simulink model "SupplyMonitor"  (R2024a)
settings: Solver=FixedStepDiscrete  StartTime=0.0  StopTime=10  FixedStep=0.01  RelTol=1e-3
model workspace (MAT data in the model file):
  CurrentInvalid_cycles = Simulink.Parameter
  CurrentInvalid_cycles.Value = 20
  CurrentInvalid_cycles.Complexity = 'real'
  CurrentInvalid_cycles.Dimensions = [1 1]
  CurrentInvalid_cycles.DataType = 'uint8'
  MinCurrentTime_cycles = Simulink.Parameter
  MinCurrentTime_cycles.Value = 20
  MinCurrentTime_cycles.Complexity = 'real'
  MinCurrentTime_cycles.Dimensions = [1 1]
  MinCurrentTime_cycles.DataType = 'uint8'
  MinCurrent_mA = Simulink.Parameter
  MinCurrent_mA.Value = 100
  MinCurrent_mA.Complexity = 'real'
  MinCurrent_mA.Dimensions = [1 1]
  MinCurrent_mA.DataType = 'single'
  OverloadHyst_mA = Simulink.Parameter
  OverloadHyst_mA.Value = 200
  OverloadHyst_mA.Complexity = 'real'
  OverloadHyst_mA.Dimensions = [1 1]
  OverloadHyst_mA.DataType = 'single'
  OverloadThd_mA = Simulink.Parameter
  OverloadThd_mA.Value = 1280
  OverloadThd_mA.Complexity = 'real'
  OverloadThd_mA.Dimensions = [1 1]
  OverloadThd_mA.DataType = 'single'
  SupplyCurrentFilter = Simulink.Parameter
  SupplyCurrentFilter.Value = 0.0078125
  SupplyCurrentFilter.Complexity = 'real'
  SupplyCurrentFilter.Dimensions = [1 1]
  SupplyCurrentFilter.DataType = 'single'
  SupplyCurrentGain = Simulink.Parameter
  SupplyCurrentGain.Value = 1
  SupplyCurrentGain.Complexity = 'real'
  SupplyCurrentGain.Dimensions = [1 1]
  SupplyCurrentGain.DataType = 'single'
values from neighbouring files (symbols this model uses):
  CurrentInvalid_cycles = 20    [SupplyMonitor_data.m]
  MinCurrent_mA = 100    [SupplyMonitor_data.m]
  MinCurrentTime_cycles = 20    [SupplyMonitor_data.m]
  OverloadHyst_mA = 200    [SupplyMonitor_data.m]
  OverloadThd_mA = 1280    [SupplyMonitor_data.m]
  SupplyCurrentFilter = 0.0078125    [SupplyMonitor_data.m]
  SupplyCurrentGain = 1.0    (= 1)    [SupplyMonitor_data.m]
undefined symbols (not defined in the file or in its folder): QLF_OK
Description:
  | 48-V-Versorgung: Strom filtern, Ueberlast mit Hysterese, LIMIT-Leitung
settings Model: ParameterArgumentNames=SupplyCurrentFilter,SupplyCurrentGain,OverloadThd_mA,OverloadHyst_mA,MinCurrent_mA,MinCurrentTime_cycles,CurrentInvalid_cycles  Creator=danie  LastModifiedBy=danie
settings OptimizationCC: DefaultParameterBehavior=Inlined  EnhancedBackFolding=on  PassReuseOutputArgsAs=Individual arguments  ZeroExternalMemoryAtStartup=off  ZeroInternalMemoryAtStartup=off  OptimizeBlockOrder=speed  DifferentSizesBufferReuse=on  OptimizationCustomize=off  EfficientTunableParamExpr=on
settings DebuggingCC: ParameterTunabilityLossMsg=error
settings HardwareCC: ProdBitPerPointer=32  ProdBitPerSizeT=32  ProdBitPerPtrDiffT=32  ProdLargestAtomicInteger=Long  ProdLargestAtomicFloat=Double  ProdWordSize=32  ProdLongLongMode=on  ProdHWDeviceType=ARM Compatible->ARM Cortex-M
settings SFSimCC: MATLABDynamicMemAlloc=off
settings RTWCC: Description=AUTOSAR  SystemTargetFile=autosar.tlc  GenCodeOnly=on  GenerateMakefile=off  TemplateMakefile=ert_default_tmf  DataTypeReplacement=CDataTypesFixedWidth
settings CodeAppCC: ForceParamTrailComments=on  IgnoreCustomStorageClasses=off  MaxIdLength=63  OperatorAnnotations=on  SimulinkDataObjDesc=on  SFDataObjDesc=on  InsertBlockDesc=on
settings STFCustomTargetCC: MultiwordLength=256  ParMdlRefBuildCompliant=on  CompOptLevelCompliant=on  IncludeMdlTerminateFcn=off  CombineOutputUpdateFcns=on  SuppressErrorStatus=on  ERTCustomFileBanners=on  SupportNonFinite=off  SupportComplex=off  SupportContinuousTime=off  SupportNonInlinedSFcns=off  RemoveResetFunc=on  MATLABClassNameForMDSCustomization=Simulink.SoftwareTarget.ERTCustomization  AutosarCompliant=on  GRTInterface=off  LookupTableObjectStructAxisOrder=2,1,3,4,...  LUTObjectStructOrderEvenSpacing=Size,Table,Breakpoints  SystemTargetFile=autosar.tlc
settings ERTTargetCC: TargetLangStandard=C99 (ISO)  ConcurrentExecutionCompliant=off  IncludeMdlTerminateFcn=off  SuppressErrorStatus=on  SupportNonFinite=off  SupportComplex=off  ModelStepFunctionPrototypeControlCompliant=off  CPPClassGenCompliant=off  AutosarCompliant=on  LookupTableObjectStructAxisOrder=2,1,3,4,...  LUTObjectStructOrderEvenSpacing=Size,Table,Breakpoints  InlinedParameterPlacement=NonHierarchical  ERTCustomFileTemplate=example_file_process.tlc  BooleanTrueId=TRUE  BooleanFalseId=FALSE

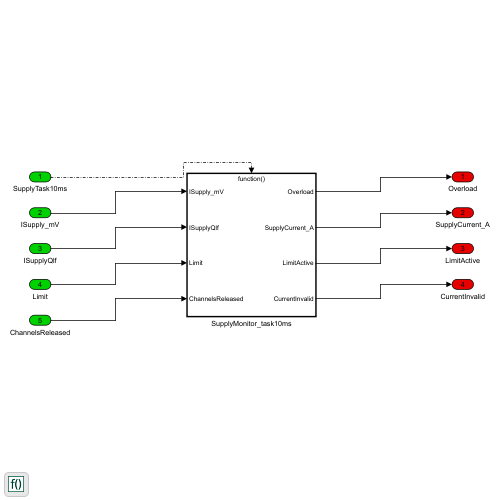
[thumbnail: Simulink's stored preview of the top-level diagram]
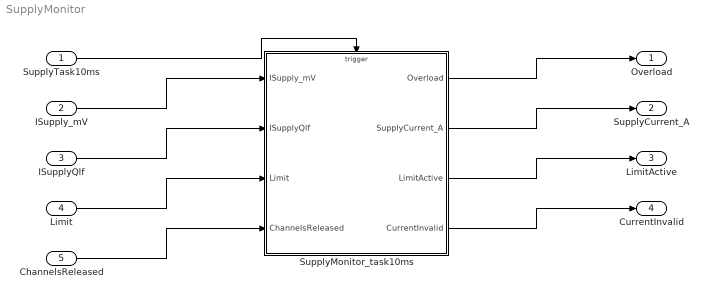
== system SupplyMonitor ==
  SupplyTask10ms : Inport  SampleTime=0.01  OutputFunctionCall=on
  ISupply_mV : Inport  Port=2  OutDataTypeStr=uint32  PortDimensions=1
  ISupplyQlf : Inport  Port=3  OutDataTypeStr=uint8  PortDimensions=1
  Limit : Inport  Port=4  OutDataTypeStr=boolean  PortDimensions=1
  ChannelsReleased : Inport  Port=5  OutDataTypeStr=boolean  PortDimensions=1
  SupplyMonitor_task10ms : Subsystem  TreatAsAtomicUnit=on
  Overload : Outport  OutDataTypeStr=boolean  PortDimensions=1
  SupplyCurrent_A : Outport  Port=2  OutDataTypeStr=single  PortDimensions=1
  LimitActive : Outport  Port=3  OutDataTypeStr=boolean  PortDimensions=1
  CurrentInvalid : Outport  Port=4  OutDataTypeStr=boolean  PortDimensions=1
  wires:
  SupplyTask10ms/1 -> SupplyMonitor_task10ms/Trigger
  ISupply_mV/1 -> SupplyMonitor_task10ms/1(ISupply_mV)
  ISupplyQlf/1 -> SupplyMonitor_task10ms/2(ISupplyQlf)
  Limit/1 -> SupplyMonitor_task10ms/3(Limit)
  ChannelsReleased/1 -> SupplyMonitor_task10ms/4(ChannelsReleased)
  SupplyMonitor_task10ms/1(Overload) -> Overload/1
  SupplyMonitor_task10ms/2(SupplyCurrent_A) -> SupplyCurrent_A/1
  SupplyMonitor_task10ms/3(LimitActive) -> LimitActive/1
  SupplyMonitor_task10ms/4(CurrentInvalid) -> CurrentInvalid/1

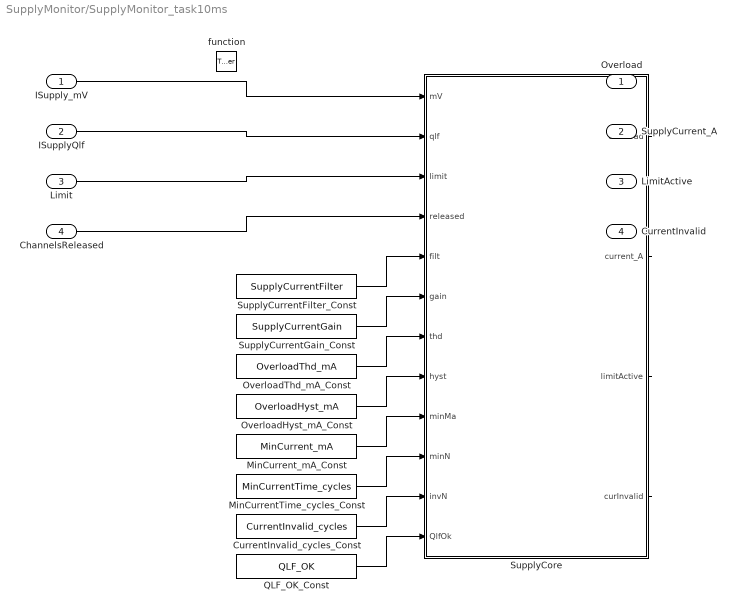
== system SupplyMonitor/SupplyMonitor_task10ms ==
  ISupply_mV : Inport
  ISupplyQlf : Inport  Port=2
  Limit : Inport  Port=3
  ChannelsReleased : Inport  Port=4
  function : TriggerPort  TriggerType=function-call  VariantControl=(inherit)  SampleTimeType=periodic  SampleTime=0.01
  CurrentInvalid_cycles_Const : Constant  Value=CurrentInvalid_cycles  OutDataTypeStr=uint8
  MinCurrentTime_cycles_Const : Constant  Value=MinCurrentTime_cycles  OutDataTypeStr=uint8
  MinCurrent_mA_Const : Constant  Value=MinCurrent_mA  OutDataTypeStr=single
  OverloadHyst_mA_Const : Constant  Value=OverloadHyst_mA  OutDataTypeStr=single
  OverloadThd_mA_Const : Constant  Value=OverloadThd_mA  OutDataTypeStr=single
  QLF_OK_Const : Constant  Value=QLF_OK  OutDataTypeStr=uint8
  SupplyCore : MATLAB Function  TreatAsAtomicUnit=on
  SupplyCurrentFilter_Const : Constant  Value=SupplyCurrentFilter  OutDataTypeStr=single
  SupplyCurrentGain_Const : Constant  Value=SupplyCurrentGain  OutDataTypeStr=single
  Overload : Outport
  SupplyCurrent_A : Outport  Port=2
  LimitActive : Outport  Port=3
  CurrentInvalid : Outport  Port=4
  wires:
  ISupply_mV/1 -> SupplyCore/1(mV)
  ISupplyQlf/1 -> SupplyCore/2(qlf)
  Limit/1 -> SupplyCore/3(limit)
  ChannelsReleased/1 -> SupplyCore/4(released)
  SupplyCurrentFilter_Const/1 -> SupplyCore/5(filt)
  SupplyCurrentGain_Const/1 -> SupplyCore/6(gain)
  OverloadThd_mA_Const/1 -> SupplyCore/7(thd)
  OverloadHyst_mA_Const/1 -> SupplyCore/8(hyst)
  MinCurrent_mA_Const/1 -> SupplyCore/9(minMa)
  MinCurrentTime_cycles_Const/1 -> SupplyCore/10(minN)
  CurrentInvalid_cycles_Const/1 -> SupplyCore/11(invN)
  QLF_OK_Const/1 -> SupplyCore/12(QlfOk)
  SupplyCore/1(overload) -> Overload/1
  SupplyCore/2(current_A) -> SupplyCurrent_A/1
  SupplyCore/3(limitActive) -> LimitActive/1
  SupplyCore/4(curInvalid) -> CurrentInvalid/1

== matlab function SupplyMonitor/SupplyMonitor_task10ms/SupplyCore ==
  data: mV input; overload output; qlf input; limit input; released input; filt input; gain input; thd input; hyst input; minMa input; minN input; invN input; QlfOk input; current_A output; limitActive output; curInvalid output
function [overload, current_A, limitActive, curInvalid] = SupplyCore(mV, qlf, limit, released, filt, gain, thd, hyst, minMa, minN, invN, QlfOk)
%SUPPLYCORE 48 V supply current filter, overload with hysteresis (see SupplyMonitor_create.m).
%#codegen
persistent y ovl bad low
if isempty(y)
    y = single(0);      % filtered current [mA]
    ovl = false;
    bad = uint8(0);     % invalid samples in a row (saturating)
    low = uint8(0);     % implausibly low valid samples in a row with a channel released (saturating)
end
if qlf == QlfOk
    sample = single(mV) * gain;
    y = y + filt * (sample - y);
    bad = uint8(0);
    if released && (sample < minMa)
        if low < uint8(255)
            low = low + uint8(1);
        end
    else
        low = uint8(0);
    end
elseif bad < uint8(255)
    bad = bad + uint8(1);
end
if ~released
    low = uint8(0);
end
if y > thd
    ovl = true;
elseif y < thd - hyst
    ovl = false;
end
overload = ovl;
c = y * single(0.001);
if c > single(65.535)
    c = single(65.535);
end
current_A = c;
limitActive = limit;
curInvalid = (bad >= invN) || (low >= minN);
